simulink model "Y3Tiltrotor_sim3_IINDI"  (R2025a)
settings: Solver=ode4  StartTime=0.0  StopTime=60  FixedStep=uavParam.sampleTime  RelTol=1e-3
PreLoadFcn:
  | filepath  = fileparts(get_param(bdroot, 'FileName'))
  | cd(filepath);
InitFcn:
  | Init_sim_IINDI;
values from neighbouring files (symbols this model uses):
  a_HOD_p = 5    [Init_sim_IINDI.m]
  a_HOD_q = 5    [Init_sim_IINDI.m]
  a_HOD_r = 5    [Init_sim_IINDI.m]
  a_HOD_u = 5    [Init_sim_IINDI.m]
  a_HOD_v = 2    [Init_sim_IINDI.m]
  a_HOD_w = 30    [Init_sim_IINDI.m]
  control = struct    [Init_sim_IINDI.m]
  env = struct    [InitData.m]
  flightState = struct    [Init_sim_IINDI.m]
  FWSpeed0 = 15    [Init_sim_IINDI.m]
  k_lpf_p = 50    [Init_sim_IINDI.m]
  k_lpf_q = 80    [Init_sim_IINDI.m]
  k_lpf_r = 100    [Init_sim_IINDI.m]
  k_lpf_u = 10    [Init_sim_IINDI.m]
  k_lpf_v = 1.5    [Init_sim_IINDI.m]
  k_lpf_w = 50    [Init_sim_IINDI.m]
  k_p = 5    [Init_sim_IINDI.m]
  k_q = 12    [Init_sim_IINDI.m]
  k_r = 0.1    [Init_sim_IINDI.m]
  k_u = 1    [Init_sim_IINDI.m]
  k_v = 0.7    [Init_sim_IINDI.m]
  k_w = 2    [Init_sim_IINDI.m]
  l_p = 30    [Init_sim_IINDI.m]
  l_q = 15    [Init_sim_IINDI.m]
  l_r = 25    [Init_sim_IINDI.m]
  l_u = 10    [Init_sim_IINDI.m]
  l_v = 1.2    [Init_sim_IINDI.m]
  l_w = 1    [Init_sim_IINDI.m]
  lamda_p = 10    [Init_sim_IINDI.m]
  lamda_q = 5    [Init_sim_IINDI.m]
  lamda_r = 1    [Init_sim_IINDI.m]
  lamda_u = 1    [Init_sim_IINDI.m]
  lamda_v = 0.15    [Init_sim_IINDI.m]
  lamda_w = 1    [Init_sim_IINDI.m]
  uavParam = struct    [InitData.m]
undefined symbols (not defined in the file or in its folder): a_HOD, a_HOD_uvw, ControlSampleTime, F, Light, MIL, Newton, Raphson
libraries: slpidlib x30, SignalEditorBlockLib x13, simulink x3, aerolibtransform2 x3, sharedtransform x3, robotcorelib x3, matrix_library x3, aerolibasang x2, aerolibutil x2, aerolibwind2 x2, shared6dof x1, aerolibatmos2 x1
(part 7 of 7)

== matlab function Y3Tiltrotor_sim3_IINDI/Subsystem/多旋翼模态/InputConditioning_stablelize/deadzone1 ==
  data: u input; y output
function y = fcn(u)
%Function description:
%  Control the range of the remote control input from RCMin to RCMax,which can be obtained from QGC. And set
%  a dead zone with a dead zone size of deadZone,the output y is normalized to 0~1.
RCMin = 1100;
RCMax = 1900;
RCMid = (RCMin + RCMax)/2;
deadZoneRate = 0.05;
deadZone = deadZoneRate*(RCMax - RCMin);
k = 1/(RCMax - RCMid - deadZone);
%Limiting
if(u < RCMin)
    u = RCMin;
elseif(u > RCMax)
    u = RCMax;
end
%dead zone and normalize
 if(u > RCMid + deadZone)
    y = (u-RCMid - deadZone)*k;
 elseif(u < RCMid - deadZone)
     y = (u - RCMid + deadZone)*k;
 else
     y = 0;
 end

 end

== matlab function Y3Tiltrotor_sim3_IINDI/Subsystem/多旋翼模态/InputConditioning_stablelize/deadzone2 ==
  data: u input; y output
function y = fcn(u)
%Function description:
%  Control the range of the remote control input from RCMin to RCMax,which can be obtained from QGC. And set
%  a dead zone with a dead zone size of deadZone,the output y is normalized to 0~1.
RCMin = 1100;
RCMax = 1900;
RCMid = (RCMin + RCMax)/2;
deadZoneRate = 0.05;
deadZone = deadZoneRate*(RCMax - RCMin);
k = 1/(RCMax - RCMid - deadZone);
%Limiting
if(u < RCMin)
    u = RCMin;
elseif(u > RCMax)
    u = RCMax;
end
%dead zone and normalize
 if(u > RCMid + deadZone)
    y = (u-RCMid - deadZone)*k;
 elseif(u < RCMid - deadZone)
     y = (u - RCMid + deadZone)*k;
 else
     y = 0;
 end

 end

== matlab function Y3Tiltrotor_sim3_IINDI/Subsystem/多旋翼模态/InputConditioning_stablelize/deadzone3 ==
  data: u input; y output
function y = fcn(u)
%Function description:
%  Control the range of the remote control input from RCMin to RCMax,which can be obtained from QGC. And set
%  a dead zone with a dead zone size of deadZone,the output y is normalized to 0~1.
RCMin = 1100;
RCMax = 1900;
RCMid = (RCMin + RCMax)/2;
deadZoneRate = 0.05;
deadZone = deadZoneRate*(RCMax - RCMin);
k = 1/(RCMax - RCMid - deadZone);
%Limiting
if(u < RCMin)
    u = RCMin;
elseif(u > RCMax)
    u = RCMax;
end
%dead zone and normalize
 if(u > RCMid + deadZone)
    y = (u-RCMid - deadZone)*k;
 elseif(u < RCMid - deadZone)
     y = (u - RCMid + deadZone)*k;
 else
     y = 0;
 end

 end

== matlab function Y3Tiltrotor_sim3_IINDI/Subsystem/多旋翼模态/Multirotor attitude control (IINDI)/Subsystem/Subsystem1/MATLAB Function ==
  settings: updateMethod=DISCRETE
  data: yaw_rate_d output; yaw_rate_desired input; yaw input; yaw_rate input; yaw_d output
function [yaw_rate_d, yaw_d] = fcn_yaw(yaw_rate_desired, yaw, yaw_rate)
% 偏航通道控制函数（与高度通道相同逻辑）
% Input:
%   yaw_rate_desired: 期望的偏航角速度（遥控器指令）
%   yaw: 当前偏航角
%   yaw_rate: 当前偏航角速度
% Output:
%   yaw_rate_d: 期望偏航角速度（传递给控制器）
%   yaw_d: 期望偏航角（传递给控制器）

persistent yaw1;
if isempty(yaw1)
    yaw1 = yaw;
end

persistent hold_yaw_flag;
if isempty(hold_yaw_flag)
    hold_yaw_flag = 0;
end

% 判断是否满足偏航锁定条件
% 条件1：期望偏航角速度很小（遥控器在中位）
% 条件2：当前偏航角速度也很小（飞行器稳定）
if abs(yaw_rate_desired) < 0.001 && abs(yaw_rate) < 0.1
    hold_yaw = 1;  % 满足锁定条件
else
    hold_yaw = 0;  % 不满足锁定条件
    hold_yaw_flag = 0;  % 重置锁定标志
end

% 首次满足锁定条件时，记录当前偏航角
% 遥控器回中且飞行器稳定时，锁定当前偏航角
if (hold_yaw > 0.5) && (hold_yaw_flag < 0.5)
    yaw1 = yaw;            % 记录当前偏航角作为锁定角度
    hold_yaw_flag = 1;     % 设置锁定标志
end

% 遥控器偏离中位，退出锁定模式
% 期望偏航角跟随当前偏航角
if hold_yaw < 0.5
    yaw1 = yaw;            % 期望偏航角 = 当前偏航角
    hold_yaw_flag = 0;     % 清除锁定标志
end

% 输出
yaw_rate_d = yaw_rate_desired;  % 直接传递期望角速度
yaw_d = yaw1;                   % 输出计算得到的期望偏航角

== matlab function Y3Tiltrotor_sim3_IINDI/Subsystem/多旋翼模态/Multirotor altitude control/Subsystem/InputConditioning_altitude/deadzone3 ==
  data: u input; y output
function y = fcn(u)
%Function description:
%  Control the range of the remote control input from RCMin to RCMax,which can be obtained from QGC. And set
%  a dead zone with a dead zone size of deadZone,the output y is normalized to 0~1.
RCMin = 1100;
RCMax = 1900;
RCMid = (RCMin + RCMax)/2;
deadZoneRate = 0.05;
deadZone = deadZoneRate*(RCMax - RCMin);
k = 1/(RCMax - RCMid - deadZone);
%Limiting
if(u < RCMin)
    u = RCMin;
elseif(u > RCMax)
    u = RCMax;
end
%dead zone and normalize
 if(u > RCMid + deadZone)
    y = (u-RCMid - deadZone)*k;
 elseif(u < RCMid - deadZone)
     y = (u - RCMid + deadZone)*k;
 else
     y = 0;
 end

 end

== matlab function Y3Tiltrotor_sim3_IINDI/Joystick and Waypoint Design/MATLAB Function2 ==
  data: ch5 input; control_mode output
function control_mode  = fcn(ch5)
%Function description:
%  Map the remote control CH5 channel to control mode
%input:
%  ch5: Remote control CH5 channel input
%  control_mode: Custom control mode
%  0: stablelize mode；1: height control mode; 2: position control mode
if ch5 < 1400
    control_mode = int8(0);
elseif ch5 < 1600
    control_mode = int8(1);
else
    control_mode = int8(2);
end

== matlab function Y3Tiltrotor_sim3_IINDI/Subsystem/多旋翼模态/Multirotor XY control/Subsystem3/InputConditioning_altitude/deadzone3 ==
  data: u input; y output
function y = fcn(u)
%Function description:
%  Control the range of the remote control input from RCMin to RCMax,which can be obtained from QGC. And set
%  a dead zone with a dead zone size of deadZone,the output y is normalized to 0~1.
RCMin = 1100;
RCMax = 1900;
RCMid = (RCMin + RCMax)/2;
deadZoneRate = 0.05;
deadZone = deadZoneRate*(RCMax - RCMin);
k = 1/(RCMax - RCMid - deadZone);
%Limiting
if(u < RCMin)
    u = RCMin;
elseif(u > RCMax)
    u = RCMax;
end
%dead zone and normalize
 if(u > RCMid + deadZone)
    y = (u-RCMid - deadZone)*k;
 elseif(u < RCMid - deadZone)
     y = (u - RCMid + deadZone)*k;
 else
     y = 0;
 end

 end

== matlab function Y3Tiltrotor_sim3_IINDI/Subsystem/多旋翼模态/MATLAB Function ==
  data: u_vy input; roll_d output
function roll_d = fcn(u_vy)

    m = 0.585;
    g = 9.81;
    
    roll_d = u_vy/(m*g);

end

== matlab function Y3Tiltrotor_sim3_IINDI/Subsystem/混控器/多旋翼混控/旋翼模态混控/Multirotor Mixer1 ==
  data: u_z input; u_phi input; u_theta input; u_psi input; u_x input; w1 output; w2 output; w3 output; Tilt1 output; Tilt2 output
function [w1,w2,w3,Tilt1,Tilt2] = fcn(u_z,u_phi,u_theta,u_psi,u_x)

    CT = 3.0123e-6;
    CQ = 4.6485e-8;
    R = 0.765;
    l = 0.2;

    if (1/(2+sqrt(3))*u_z-0.5*u_phi+sqrt(3)/(4+2*sqrt(3))*u_theta) == 0
        Tilt1_bar = 0;
    else
        Tilt1_bar = atan((CQ*R/(CT*l)*u_phi-1/l*u_psi+0.5*u_x)/(1/(2+sqrt(3))*u_z-0.5*u_phi+sqrt(3)/(4+2*sqrt(3))*u_theta));
    end
    if Tilt1_bar >= 45*pi/180
        Tilt1 = 45*pi/180;
    elseif Tilt1_bar <= -15*pi/180
        Tilt1 = -15*pi/180;
    else
        Tilt1 = Tilt1_bar;
    end

    if (1/(2+sqrt(3))*u_z+0.5*u_phi+sqrt(3)/(4+2*sqrt(3))*u_theta) == 0
        Tilt2_bar = 0;
    else
        Tilt2_bar = atan((-CQ*R/(CT*l)*u_phi+1/l*u_psi+0.5*u_x)/(1/(2+sqrt(3))*u_z+0.5*u_phi+sqrt(3)/(4+2*sqrt(3))*u_theta));
    end
    if Tilt2_bar >= 45*pi/180
        Tilt2 = 45*pi/180;
    elseif Tilt2_bar <= -15*pi/180
        Tilt2 = -15*pi/180;
    else
        Tilt2 = Tilt2_bar;
    end

    w1 = ((1/(2+sqrt(3)))*u_z - (1/2)*u_phi + (sqrt(3)/(4+2*sqrt(3)))*u_theta)/cos(Tilt1);
    w2 = ((1/(2+sqrt(3)))*u_z + (1/2)*u_phi + (sqrt(3)/(4+2*sqrt(3)))*u_theta)/cos(Tilt2);
    w3 = (sqrt(3)/(2+sqrt(3)))*u_z - (sqrt(3)/(2+sqrt(3)))*u_theta;

end

== matlab function Y3Tiltrotor_sim3_IINDI/Subsystem/混控器/多旋翼混控/旋翼模态混控/Multirotor Mixer4 (对应论文) ==
  data: u_z input; u_phi input; u_theta input; u_psi input; u_x input; w1 output; w2 output; w3 output; Tilt1 output; Tilt2 output
function [w1,w2,w3,Tilt1,Tilt2] = fcn(u_z,u_phi,u_theta,u_psi,u_x)
    
    CT = 9.5883e-7;
    CQ = 1.4797e-8;
    R = 0.765;
    l1 = 0.13;
    l2 = 0.24;

    k = (CQ*R)/CT;

    G = [0   1  0  1  1;
         k -l1 -k l1  0;
         0  l1  0 l1 -l2;
        -l1 -k l1  k  0;
         1  0   1  0  0];
    G_inv = inv(G);

    u = [u_z,u_phi,u_theta,u_psi,u_x]';
    u_act = G_inv*u;

    if u_act(2) == 0
        Tilt1_bar = 0;
    else
        Tilt1_bar = atan(u_act(1)/u_act(2));
    end
    if Tilt1_bar >= 45*pi/180
        Tilt1 = 45*pi/180;
    elseif Tilt1_bar <= -15*pi/180
        Tilt1 = -15*pi/180;
    else
        Tilt1 = Tilt1_bar;
    end

    if u_act(4) == 0
        Tilt2_bar = 0;
    else
        Tilt2_bar = atan(u_act(3)/u_act(4));
    end
    if Tilt2_bar >= 45*pi/180
        Tilt2 = 45*pi/180;
    elseif Tilt2_bar <= -15*pi/180
        Tilt2 = -15*pi/180;
    else
        Tilt2 = Tilt2_bar;
    end

    w1_bar = u_act(2)/cos(Tilt1);
    if w1_bar <= 0
        w1 = 0;
    else
        w1 = w1_bar;
    end

    w2_bar = u_act(4)/cos(Tilt2);
    if w2_bar <= 0
        w2 = 0;
    else
        w2 = w2_bar;
    end

    w3_bar = u_act(5);
    if w3_bar <= 0
        w3 = 0;
    else
        w3 = w3_bar;
    end

end

== matlab function Y3Tiltrotor_sim3_IINDI/Joystick and Waypoint Design/MATLAB Function ==
  data: t input; x_ref output; y_ref output; z_ref output; psi_ref output; theta_ref output
function [x_ref, y_ref, z_ref, psi_ref, theta_ref] = generate_trajectory_fixed_yaw(t)
% 生成8字形轨迹（固定偏航角）
% 输入：当前时间 t（秒）
% 输出：期望位置x,y,z和偏航角psi

% 参数定义
T_takeoff = 20;     % 起飞阶段持续时间（秒）
H_cruise = 50;      % 巡航高度（米）
A = 10;              % 8字形x方向振幅（米）
B = 8;              % 8字形y方向振幅（米）
omega = 0.2;        % 角频率（rad/s）
circles = 3;         % 8字形飞行圈数
T_circle = 2*pi/omega; % 单圈周期（秒）
T_cruise = circles * T_circle; % 巡航总时间
T_land = 20;         % 降落阶段持续时间（秒）

% 计算任务总时间和各阶段时间点
T_total = T_takeoff + T_cruise + T_land;
t_cruise_start = T_takeoff;
t_land_start = T_takeoff + T_cruise;

% 偏航角固定为0（朝北）
psi_fixed = 0;

    % 起飞阶段（0 ≤ t < T_takeoff）
    if t < T_takeoff
        % 垂直起飞
        x_ref = 0;
        y_ref = 0;
        z_ref = (t / T_takeoff) * H_cruise;  % 线性上升
        psi_ref = psi_fixed;
        theta_ref = 0;
        
    elseif t < t_land_start
        % 8字形轨迹阶段
        t_cruise = t - t_cruise_start;
        
        % 8字形参数方程（Lemniscate of Bernoulli）
        % 使用改进的8字形方程，避免奇点
        theta = omega * t_cruise;
        
        % 方法1：使用椭圆8字形
        x_ref = A * sin(theta);
        y_ref = B * sin(2 * theta) / 2;
        
        % 方法2：使用更平滑的8字形（可选）
        % r = sqrt(cos(2*theta) + sqrt(1.1 - sin(2*theta)^2));
        % x_ref = A * r * cos(theta);
        % y_ref = B * r * sin(theta);
        
        z_ref = H_cruise;
        psi_ref = psi_fixed;
        theta_ref = 0;
    
    elseif t < T_total
        % 计算降落阶段的时间
        t_land = t - t_land_start;
        tau = t_land / T_land;
        
        % 平滑过渡到降落（使用五次多项式）
        % 从8字形的结束位置平滑回到原点
        theta_end = omega * T_cruise;
        x_end = A * sin(theta_end);
        y_end = B * sin(2 * theta_end) / 2;
        
        % 位置从8字形结束点平滑回到原点
        x_ref = x_end * (1 - tau);
        y_ref = y_end * (1 - tau);
        
        % 高度平滑下降（从H_cruise到0）
        z_ref = H_cruise * (1 - tau);
        psi_ref = psi_fixed;
        theta_ref = 0;
    
    else
        x_ref = 0;
        y_ref = 0;
        z_ref = 0;
        psi_ref = psi_fixed;
        theta_ref = 0;
    end



end

== matlab function Y3Tiltrotor_sim3_IINDI/Subsystem/固定翼模态/InputConditioning_stablelize/deadzone0 ==
  data: u input; y output
function y = fcn(u)
%Function description:
%  Control the range of the remote control input from RCMin to RCMax,which can be obtained from QGC. And set
%  a dead zone with a dead zone size of deadZone,the output y is normalized to 0~1.
RCMin = 1100;
RCMax = 1900;
RCMid = (RCMin + RCMax)/2;
deadZoneRate = 0.05;
deadZone = deadZoneRate*(RCMax - RCMin);
k = 1/(RCMax - RCMid - deadZone);
%Limiting
if(u < RCMin)
    u = RCMin;
elseif(u > RCMax)
    u = RCMax;
end
%dead zone and normalize
 if(u > RCMid + deadZone)
    y = (u-RCMid - deadZone)*k;
 elseif(u < RCMid - deadZone)
     y = (u - RCMid + deadZone)*k;
 else
     y = 0;
 end

 end

== matlab function Y3Tiltrotor_sim3_IINDI/Y3 Tiltrotor Aircraft Model/Subsystem/Aerodynamic Forces and Moments/Compute Body Frame Aerodynamic Forces and Moments/Wind frame F& M/Longitudinal Channel/CL/CL(delta_e) ==
  data: delta_e input; CL_delta_e output
function CL_delta_e = fcn_CL_delta_e(delta_e)

    c1 = 0.000343;
    c2 = 47.4;
    c3 = -11.336446;
    c4 = -0.081703;
    c5 = -0.548177;
    c6 = -0.772571;
    c7 = 25.051196;

    CL_delta_e = (1+tanh(c1*(c2^2-delta_e.^2)))/(1+tanh(c1*c2^2)).*(c3*sin(c4*pi/180*delta_e))...
            +(1-(1+tanh(c1*(c2^2-delta_e.^2)))/(1+tanh(c1*c2^2))).*(c5*sin(c6*pi/180*delta_e+c7));
    
end

== matlab function Y3Tiltrotor_sim3_IINDI/Subsystem/固定翼模态/InputConditioning_stablelize/deadzone1 ==
  data: u input; y output
function y = fcn(u)
%Function description:
%  Control the range of the remote control input from RCMin to RCMax,which can be obtained from QGC. And set
%  a dead zone with a dead zone size of deadZone,the output y is normalized to 0~1.
RCMin = 1100;
RCMax = 1900;
RCMid = (RCMin + RCMax)/2;
deadZoneRate = 0.05;
deadZone = deadZoneRate*(RCMax - RCMin);
k = 1/(RCMax - RCMid - deadZone);
%Limiting
if(u < RCMin)
    u = RCMin;
elseif(u > RCMax)
    u = RCMax;
end
%dead zone and normalize
 if(u > RCMid + deadZone)
    y = (u-RCMid - deadZone)*k;
 elseif(u < RCMid - deadZone)
     y = (u - RCMid + deadZone)*k;
 else
     y = 0;
 end

 end

== matlab function Y3Tiltrotor_sim3_IINDI/Subsystem/固定翼模态/InputConditioning_stablelize/deadzone2 ==
  data: u input; y output
function y = fcn(u)
%Function description:
%  Control the range of the remote control input from RCMin to RCMax,which can be obtained from QGC. And set
%  a dead zone with a dead zone size of deadZone,the output y is normalized to 0~1.
RCMin = 1100;
RCMax = 1900;
RCMid = (RCMin + RCMax)/2;
deadZoneRate = 0.05;
deadZone = deadZoneRate*(RCMax - RCMin);
k = 1/(RCMax - RCMid - deadZone);
%Limiting
if(u < RCMin)
    u = RCMin;
elseif(u > RCMax)
    u = RCMax;
end
%dead zone and normalize
 if(u > RCMid + deadZone)
    y = (u-RCMid - deadZone)*k;
 elseif(u < RCMid - deadZone)
     y = (u - RCMid + deadZone)*k;
 else
     y = 0;
 end

 end

== matlab function Y3Tiltrotor_sim3_IINDI/Subsystem/固定翼模态/InputConditioning_stablelize/deadzone3 ==
  data: u input; y output
function y = fcn(u)
%Function description:
%  Control the range of the remote control input from RCMin to RCMax,which can be obtained from QGC. And set
%  a dead zone with a dead zone size of deadZone,the output y is normalized to 0~1.
RCMin = 1000;
RCMax = 2000;
RCMid = (RCMin + RCMax)/2;
deadZoneRate = 0.05;
deadZone = deadZoneRate*(RCMax - RCMin);
k = 1/(RCMax - RCMid - deadZone);
%Limiting
if(u < RCMin)
    u = RCMin;
elseif(u > RCMax)
    u = RCMax;
end
%dead zone and normalize
 if(u > RCMid + deadZone)
    y = (u-RCMid - deadZone)*k;
 elseif(u < RCMid - deadZone)
     y = (u - RCMid + deadZone)*k;
 else
     y = 0;
 end

 end

== matlab function Y3Tiltrotor_sim3_IINDI/Subsystem/固定翼模态/InputConditioning_altitude/deadzone3 ==
  data: u input; y output
function y = fcn(u)
%Function description:
%  Control the range of the remote control input from RCMin to RCMax,which can be obtained from QGC. And set
%  a dead zone with a dead zone size of deadZone,the output y is normalized to 0~1.
RCMin = 1100;
RCMax = 1900;
RCMid = (RCMin + RCMax)/2;
deadZoneRate = 0.05;
deadZone = deadZoneRate*(RCMax - RCMin);
k = 1/(RCMax - RCMid - deadZone);
%Limiting
if(u < RCMin)
    u = RCMin;
elseif(u > RCMax)
    u = RCMax;
end
%dead zone and normalize
 if(u > RCMid + deadZone)
    y = (u-RCMid - deadZone)*k;
 elseif(u < RCMid - deadZone)
     y = (u - RCMid + deadZone)*k;
 else
     y = 0;
 end

 end

== matlab function Y3Tiltrotor_sim3_IINDI/Subsystem/固定翼模态/InputConditioning_speed/deadzone3 ==
  data: u input; y output
function y = fcn(u)
%Function description:
%  Control the range of the remote control input from RCMin to RCMax,which can be obtained from QGC. And set
%  a dead zone with a dead zone size of deadZone,the output y is normalized to 0~1.
RCMin = 1100;
RCMax = 1900;
RCMid = (RCMin + RCMax)/2;
deadZoneRate = 0.05;
deadZone = deadZoneRate*(RCMax - RCMin);
k = 1/(RCMax - RCMid - deadZone);
%Limiting
if(u < RCMin)
    u = RCMin;
elseif(u > RCMax)
    u = RCMax;
end
%dead zone and normalize
 if(u > RCMid + deadZone)
    y = (u-RCMid - deadZone)*k;
 elseif(u < RCMid - deadZone)
     y = (u - RCMid + deadZone)*k;
 else
     y = 0;
 end

 end

== matlab function Y3Tiltrotor_sim3_IINDI/Subsystem/固定翼模态/高度-速度控制/定速模式/TECS/MATLAB Function ==
  data: Airspeed input; V output
function V = fcn(Airspeed)

    if abs(Airspeed) <= 0.001
        V = 0.001;
    else
        V = Airspeed;
    end

end

== matlab function Y3Tiltrotor_sim3_IINDI/Subsystem/固定翼模态/高度-速度控制/定速模式/Subsystem1/Subsystem/InputConditioning_altitude/MATLAB Function ==
  data: u input; vz_cmd output; z_e input
function vz_cmd = fcn(u,z_e)

    if z_e >= -0.001 && u < 0 
        vz_cmd = 0;
    else
        vz_cmd = u;
    end

end

== matlab function Y3Tiltrotor_sim3_IINDI/Subsystem/固定翼模态/高度-速度控制/定高模式/Subsystem/InputConditioning_altitude/MATLAB Function ==
  data: u input; vz_cmd output; z_e input
function vz_cmd = fcn(u,z_e)

    if z_e >= -0.001 && u < 0 
        vz_cmd = 0;
    else
        vz_cmd = u;
    end

end

== matlab function Y3Tiltrotor_sim3_IINDI/Subsystem/多旋翼模态/Multirotor XY control1/Subsystem/InputConditioning_altitude/deadzone3 ==
  data: u input; y output
function y = fcn(u)
%Function description:
%  Control the range of the remote control input from RCMin to RCMax,which can be obtained from QGC. And set
%  a dead zone with a dead zone size of deadZone,the output y is normalized to 0~1.
RCMin = 1100;
RCMax = 1900;
RCMid = (RCMin + RCMax)/2;
deadZoneRate = 0.05;
deadZone = deadZoneRate*(RCMax - RCMin);
k = 1/(RCMax - RCMid - deadZone);
%Limiting
if(u < RCMin)
    u = RCMin;
elseif(u > RCMax)
    u = RCMax;
end
%dead zone and normalize
 if(u > RCMid + deadZone)
    y = (u-RCMid - deadZone)*k;
 elseif(u < RCMid - deadZone)
     y = (u - RCMid + deadZone)*k;
 else
     y = 0;
 end

 end

== matlab function Y3Tiltrotor_sim3_IINDI/Subsystem/多旋翼模态/Multirotor XY control1/Subsystem3/InputConditioning_altitude/deadzone3 ==
  data: u input; y output
function y = fcn(u)
%Function description:
%  Control the range of the remote control input from RCMin to RCMax,which can be obtained from QGC. And set
%  a dead zone with a dead zone size of deadZone,the output y is normalized to 0~1.
RCMin = 1100;
RCMax = 1900;
RCMid = (RCMin + RCMax)/2;
deadZoneRate = 0.05;
deadZone = deadZoneRate*(RCMax - RCMin);
k = 1/(RCMax - RCMid - deadZone);
%Limiting
if(u < RCMin)
    u = RCMin;
elseif(u > RCMax)
    u = RCMax;
end
%dead zone and normalize
 if(u > RCMid + deadZone)
    y = (u-RCMid - deadZone)*k;
 elseif(u < RCMid - deadZone)
     y = (u - RCMid + deadZone)*k;
 else
     y = 0;
 end

 end

== matlab function Y3Tiltrotor_sim3_IINDI/Y3 Tiltrotor Aircraft Model/Subsystem/Aerodynamic Forces and Moments/Compute Body Frame Aerodynamic Forces and Moments/Wind frame F& M/Longitudinal Channel/CL/CL(alpha) ==
  data: CL_alpha output; alpha input
function CL_alpha = piecewise_CL_alpha(alpha)

    c1 = 51.38;
    c2 = 18.4;
    c3 = 0.106096;
    c4 = -0.999417;
    c5 = -3.039833;
    c6 = -0.864898;
    c7 = 0.956252;
    c8 = -1.573247;
    c9 = 5.019980;
    c10 = 14.998103;
    c11 = 0.619631;
    c12 = 1.474257;
    c13 = 5.709070;

    CL_alpha = zeros(size(alpha));

    idx_pos = alpha >= 0;
    if any(idx_pos)
        alpha_pos = alpha(idx_pos);
        CL_alpha(idx_pos) = (1+tanh(c1*(c2^2-alpha_pos.^2)))/(1+tanh(c1*c2^2)).*(c3+c4*sin(c5*pi/180*alpha_pos))...
            +(1-(1+tanh(c1*(c2^2-alpha_pos.^2)))/(1+tanh(c1*c2^2))).*(c6*sin(c7*pi/180*alpha_pos+c8));
    end
    
    idx_neg = alpha < 0;
    if any(idx_neg)
        alpha_neg = alpha(idx_neg);
        CL_alpha(idx_neg) = (1+tanh(c9*(c10^2-alpha_neg.^2)))/(1+tanh(c9*c10^2)).*(c3+c4*sin(c5*pi/180*alpha_neg))...
            +(1-(1+tanh(c9*(c10^2-alpha_neg.^2)))/(1+tanh(c9*c10^2))).*(c11*sin(c12*pi/180*alpha_neg+c13));
    end

end

== matlab function Y3Tiltrotor_sim3_IINDI/Y3 Tiltrotor Aircraft Model/States Bus/MATLAB Function1 ==
  data: vxyz input; course output; gndSpeed output
function [course, gndSpeed] = fcn(vxyz)

vx = vxyz(1);
vy = vxyz(2);
course = atan2(vy, vx);
gndSpeed = norm([vx vy 0]);

== matlab function Y3Tiltrotor_sim3_IINDI/Y3 Tiltrotor Aircraft Model/Subsystem/Aerodynamic Forces and Moments/Compute Body Frame Aerodynamic Forces and Moments/Wind frame F& M/Longitudinal Channel/CD/CD(alpha) ==
  data: alpha input; CD_alpha output
function CD_alpha = piecewise_CD_alpha(alpha)

    c1 = 10.5;
    c2 = 0.023013;
    c3 = 0.000398;
    c4 = 1.077953;
    c5 = -1.061505;
    c6 = 0.919668;
    c7 = -7.769775;
    c8 = 49.988;
    c9 = -0.043323;
    c10 = 1.088698;
    c11 = 0.891002;
    c12 = -9.586878;

    CD_alpha = zeros(size(alpha));

    idx_pos = alpha >= 0;
    if any(idx_pos)
        alpha_pos = alpha(idx_pos);
        CD_alpha(idx_pos) = (1+tanh(c1*(18.4^2-alpha_pos.^2)))/(1+tanh(c1*18.4^2)).*(c2+c3*alpha_pos.^2)...
            +(1-(1+tanh(c1*(18.4^2-alpha_pos.^2)))/(1+tanh(c1*18.4^2))).*(c4+c5*sin(c6*pi/180*alpha_pos+c7).^2);
    end
    
    idx_neg = alpha < 0;
    if any(idx_neg)
        alpha_neg = alpha(idx_neg);
        CD_alpha(idx_neg) = (1+tanh(c8*(15^2-alpha_neg.^2)))/(1+tanh(c8*15^2)).*(c2+c3*alpha_neg.^2)...
            +(1-(1+tanh(c8*(15^2-alpha_neg.^2)))/(1+tanh(c8*15^2))).*(c9+c10*sin(c11*pi/180*alpha_neg+c12).^2);
    end

end

== matlab function Y3Tiltrotor_sim3_IINDI/Y3 Tiltrotor Aircraft Model/Subsystem/Aerodynamic Forces and Moments/Compute Body Frame Aerodynamic Forces and Moments/Wind frame F& M/Longitudinal Channel/Cm/Cm(alpha) ==
  data: Cm_alpha output; alpha input
function Cm_alpha = piecewise_Cm_alpha(alpha)

    c1 = 0.000219;
    c2 = -0.011442;
    c3 = 0.056866;
    c4 = -3.422369;
    c5 = -1.763366;
    c6 = -0.059447;
    c7 = 3.052526;
    c8 = 0.000256;
    c9 = -3.005585;
    c10 = -0.035985;
    c11 = -15.643618;

    Cm_alpha = zeros(size(alpha));

    idx_pos = alpha >= 0;
    if any(idx_pos)
        alpha_pos = alpha(idx_pos);
        Cm_alpha(idx_pos) = (1+tanh(c1*(18.4^2-alpha_pos.^2)))/(1+tanh(c1*18.4^2)).*(c2+c3*sin(c4*pi/180*alpha_pos))...
            +(1-(1+tanh(c1*(18.4^2-alpha_pos.^2)))/(1+tanh(c1*18.4^2))).*(c5*sin(c6*pi/180*alpha_pos+c7));
    end
    
    idx_neg = alpha < 0;
    if any(idx_neg)
        alpha_neg = alpha(idx_neg);
        Cm_alpha(idx_neg) = (1+tanh(c8*(15^2-alpha_neg.^2)))/(1+tanh(c8*15^2)).*(c2+c3*sin(c4*pi/180*alpha_neg))...
            +(1-(1+tanh(c8*(15^2-alpha_neg.^2)))/(1+tanh(c8*15^2))).*(c9*sin(c10*pi/180*alpha_neg+c11));
    end

end

== matlab function Y3Tiltrotor_sim3_IINDI/Y3 Tiltrotor Aircraft Model/Subsystem/Aerodynamic Forces and Moments/Compute Body Frame Aerodynamic Forces and Moments/Wind frame F& M/Lateral Channel/CY/CY(beta) ==
  data: CY_beta output; beta input
function CY_beta = fcn_CY_beta(beta)

    c1 = 65.424349;
    c2 = 41.5;
    c3 = 0.100430;
    c4 = -1.744107;
    c5 = 0.083409;
    c6 = 1.914772;
    c7 = -3.141796;

    CY_beta = (1+tanh(c1*(c2^2-beta.^2)))/(1+tanh(c1*c2^2)).*(c3*sin(c4*pi/180*beta))...
        + (1-(1+tanh(c1*(c2^2-beta.^2)))/(1+tanh(c1*c2^2))).*(c5*sin(c6*pi/180*beta+c7));

end

== matlab function Y3Tiltrotor_sim3_IINDI/Y3 Tiltrotor Aircraft Model/Subsystem/Aerodynamic Forces and Moments/Compute Body Frame Aerodynamic Forces and Moments/Wind frame F& M/Lateral Channel/Cl/Cl(beta) ==
  data: Cl1_beta output; beta input
function Cl1_beta = fcn_Cl1_beta(beta)

    c1 = 18.339628;
    c2 = 41.5;
    c3 = 0.035354;
    c4 = -1.788085;
    c5 = 0.035299;
    c6 = -1.515415;
    c7 = 0.001573;

    Cl1_beta = (1+tanh(c1*(c2^2-beta.^2)))/(1+tanh(c1*c2^2)).*(c3*sin(c4*pi/180*beta))...
        + (1-(1+tanh(c1*(c2^2-beta.^2)))/(1+tanh(c1*c2^2))).*(c5*sin(c6*pi/180*beta+c7));

end

== matlab function Y3Tiltrotor_sim3_IINDI/Y3 Tiltrotor Aircraft Model/Subsystem/Aerodynamic Forces and Moments/Compute Body Frame Aerodynamic Forces and Moments/Wind frame F& M/Lateral Channel/Cn/Cn(beta) ==
  data: Cn_beta output; beta input
function Cn_beta = fcn_Cn_beta(beta)

    c1 = 16.018126;
    c2 = 41.5;
    c3 = 0.045296;
    c4 = 0.918923;
    c5 = 0.028417;
    c6 = 1.203453;
    c7 = 6.274968;

    Cn_beta = (1+tanh(c1*(c2^2-beta.^2)))/(1+tanh(c1*c2^2)).*(c3*sin(c4*pi/180*beta))...
        + (1-(1+tanh(c1*(c2^2-beta.^2)))/(1+tanh(c1*c2^2))).*(c5*sin(c6*pi/180*beta+c7));

end

== matlab function Y3Tiltrotor_sim3_IINDI/Y3 Tiltrotor Aircraft Model/Subsystem/Aerodynamic Forces and Moments/Compute Body Frame Aerodynamic Forces and Moments/Wind frame F& M/Longitudinal Channel/Cm/Cm(delta_e) ==
  data: delta_e input; Cm_delta_e output
function Cm_delta_e = fcn_Cm_delta_e(delta_e)

    c1 = 0.000301;
    c2 = -1.724970;
    c3 = 0.142608;
    c4 = 0.109046;
    c5 = 0.694663;
    c6 = -2.968985;

    Cm_delta_e = (1+tanh(c1*(47.5^2-delta_e.^2)))/(1+tanh(c1*47.5^2)).*(c2*sin(c3*pi/180*delta_e))...
            +(1-(1+tanh(c1*(47.5^2-delta_e.^2)))/(1+tanh(c1*47.5^2))).*(c4*sin(c5*pi/180*delta_e+c6));

end

== matlab function Y3Tiltrotor_sim3_IINDI/Y3 Tiltrotor Aircraft Model/Subsystem/Aerodynamic Forces and Moments/Compute Body Frame Aerodynamic Forces and Moments/Wind frame F& M/Longitudinal Channel/CD/CD(delta_e) ==
  data: delta_e input; CD_delta_e output
function CD_delta_e = fcn_CD_delta_e(delta_e)

    c1 = 0.000707;
    c2 = 0.000057;
    c3 = 0.013601;
    c4 = 0.101850;
    c5 = 1.443831;
    c6 = 56.012704;
    c7 = 0.000024;
    c8 = 0.101300;
    c9 = -0.021731;
    c10 = -3.024408;
    c11 = 61.266062;

    CD_delta_e = zeros(size(delta_e));

    idx_pos = delta_e >= 0;
    if any(idx_pos)
        delta_e_pos = delta_e(idx_pos);
        CD_delta_e(idx_pos) = (1+tanh(c1*(47.4^2-delta_e_pos.^2)))/(1+tanh(c1*47.4^2)).*(c2*delta_e_pos.^2)...
            +(1-(1+tanh(c1*(47.4^2-delta_e_pos.^2)))/(1+tanh(c1*47.4^2))).*(c3+c4*sin(c5*pi/180*delta_e_pos+c6).^2);
    end

    idx_neg = delta_e < 0;
    if any(idx_neg)
        delta_e_neg = delta_e(idx_neg);
        CD_delta_e(idx_neg) = (1+tanh(c1*(47.4^2-delta_e_neg.^2)))/(1+tanh(c1*47.4^2)).*(c7*delta_e_neg.^2)...
            +(1-(1+tanh(c1*(47.4^2-delta_e_neg.^2)))/(1+tanh(c1*47.4^2))).*(c8+c9*sin(c10*pi/180*delta_e_neg+c11).^2);
    end
    
end
